simulink model "AXU5EV_Experiment_FOC"  (R2026b)
settings: Solver=FixedStepDiscrete  StopTime=.01  FixedStep=Ts_ACR
model workspace (MAT data in the model file):
  ADC_Calibration_Log2_N = 10
  ADC_Manual_Offset_Valid_A = 0
  ADC_Manual_Offset_Valid_B = 0
  Encoder_Counts_Per_Electrical_Period = 30000
  Encoder_Nanometres_Per_Count = 1000
  Experiment_Id_Limit_A = 0.5
  Experiment_Iq_Limit_A = 0.3
  Experiment_Parameter_Version = 20261117
  FOC_Fixed_Config.Version = 20261024
  FOC_Fixed_Config.Parameters.Rs = 1.45
  FOC_Fixed_Config.Parameters.Ld = 0.0118
  FOC_Fixed_Config.Parameters.Lq = 0.0118
  FOC_Fixed_Config.Parameters.psi = 0.0684240400279
  FOC_Fixed_Config.Parameters.Kp_ACR = 59
  FOC_Fixed_Config.Parameters.Ki_ACR = 7250
  FOC_Fixed_Config.Parameters.Kaw_d = 0.0122881355932
  FOC_Fixed_Config.Parameters.Kaw_q = 0.0122881355932
  FOC_Fixed_Config.Parameters.Ts_ACR = 0.0001
  FOC_Fixed_Config.Parameters.Udc = 48
  FOC_Fixed_Config.Fimath = embedded.fimath
  FOC_Fixed_Config.Fimath.RoundMode = 'convergent'
  FOC_Fixed_Config.Fimath.RoundingMethod = 'Convergent'
  FOC_Fixed_Config.Fimath.OverflowMode = 'saturate'
  FOC_Fixed_Config.Fimath.OverflowAction = 'Saturate'
  FOC_Fixed_Config.Fimath.ProductMode = 'FullPrecision'
  FOC_Fixed_Config.Fimath.SumMode = 'FullPrecision'
  FOC_Fixed_Config.Fimath.FixedOpFloatingYields = 'Fixed'
  FOC_Fixed_Config.Fimath.ProductWordLength = 32
  FOC_Fixed_Config.Fimath.SumWordLength = 32
  FOC_Fixed_Config.Fimath.MaxProductWordLength = 65535
  FOC_Fixed_Config.Fimath.MaxSumWordLength = 65535
  FOC_Fixed_Config.Fimath.ProductFractionLength = 30
  FOC_Fixed_Config.Fimath.ProductFixedExponent = -30
  FOC_Fixed_Config.Fimath.SumFractionLength = 30
  FOC_Fixed_Config.Fimath.SumFixedExponent = -30
  FOC_Fixed_Config.Fimath.SumSlopeAdjustmentFactor = 1
  FOC_Fixed_Config.Fimath.SumBias = 0
  FOC_Fixed_Config.Fimath.ProductSlopeAdjustmentFactor = 1
  FOC_Fixed_Config.Fimath.ProductBias = 0
  FOC_Fixed_Config.Fimath.CastBeforeSum = 1
  FOC_Fixed_Config.Fimath.SumSlope = 9.31322574615e-10
  FOC_Fixed_Config.Fimath.ProductSlope = 9.31322574615e-10
  FOC_Fixed_Config.Fimath.DDGMaxProductWordLength = 65535
  FOC_Fixed_Config.Fimath.DDGMaxSumWordLength = 65535
  FOC_Fixed_Config.Fimath.DDGProductFixedExponent = -30
  FOC_Fixed_Config.Fimath.DDGProductFractionLength = 30
  FOC_Fixed_Config.Fimath.DDGProductWordLength = 32
  FOC_Fixed_Config.Fimath.DDGSumFixedExponent = -30
  FOC_Fixed_Config.Fimath.DDGSumFractionLength = 30
  FOC_Fixed_Config.Fimath.DDGSumWordLength = 32
  FOC_Fixed_Config.Fimath.DDGProductBias = 0
  FOC_Fixed_Config.Fimath.DDGProductSlopeAdjustmentFactor = 1
  FOC_Fixed_Config.Fimath.DDGSumBias = 0
  FOC_Fixed_Config.Fimath.DDGSumSlopeAdjustmentFactor = 1
  FOC_Fixed_Config.Fimath.DDGCastBeforeSum = 1
  FOC_Fixed_Config.Fimath.DDGProductSlope = 9.31322574615e-10
  FOC_Fixed_Config.Fimath.DDGSumSlope = 9.31322574615e-10
  FOC_Fixed_Config.Types.Current = embedded.numerictype
  FOC_Fixed_Config.Types.Current.ReadOnly = 0
  FOC_Fixed_Config.Types.Current.Volatile = 0
  FOC_Fixed_Config.Types.Current.DataTypeMode = 'Fixed-point: binary point scaling'
  FOC_Fixed_Config.Types.Current.DataType = 'Fixed'
  FOC_Fixed_Config.Types.Current.Scaling = 'BinaryPoint'
  FOC_Fixed_Config.Types.Current.SignednessBool = 1
  FOC_Fixed_Config.Types.Current.Signedness = 'Signed'
  FOC_Fixed_Config.Types.Current.Signed = 1
  FOC_Fixed_Config.Types.Current.WordLength = 32
  FOC_Fixed_Config.Types.Current.FractionLength = 24
  FOC_Fixed_Config.Types.Current.BinaryPoint = 24
  FOC_Fixed_Config.Types.Current.Slope = 5.96046447754e-08
  FOC_Fixed_Config.Types.Current.FixedExponent = -24
  FOC_Fixed_Config.Types.Current.SlopeAdjustmentFactor = 1
  FOC_Fixed_Config.Types.Current.Bias = 0
  FOC_Fixed_Config.Types.Current.DataTypeOverride = 'Inherit'
  FOC_Fixed_Config.Types.Angle = embedded.numerictype
  FOC_Fixed_Config.Types.Angle.ReadOnly = 0
  FOC_Fixed_Config.Types.Angle.Volatile = 0
  FOC_Fixed_Config.Types.Angle.DataTypeMode = 'Fixed-point: binary point scaling'
  FOC_Fixed_Config.Types.Angle.DataType = 'Fixed'
  FOC_Fixed_Config.Types.Angle.Scaling = 'BinaryPoint'
  FOC_Fixed_Config.Types.Angle.SignednessBool = 1
  FOC_Fixed_Config.Types.Angle.Signedness = 'Signed'
  FOC_Fixed_Config.Types.Angle.Signed = 1
  FOC_Fixed_Config.Types.Angle.WordLength = 40
  FOC_Fixed_Config.Types.Angle.FractionLength = 32
  FOC_Fixed_Config.Types.Angle.BinaryPoint = 32
  FOC_Fixed_Config.Types.Angle.Slope = 2.32830643654e-10
  FOC_Fixed_Config.Types.Angle.FixedExponent = -32
  FOC_Fixed_Config.Types.Angle.SlopeAdjustmentFactor = 1
  FOC_Fixed_Config.Types.Angle.Bias = 0
  FOC_Fixed_Config.Types.Angle.DataTypeOverride = 'Inherit'
  FOC_Fixed_Config.Types.Omega = embedded.numerictype
  FOC_Fixed_Config.Types.Omega.ReadOnly = 0
  FOC_Fixed_Config.Types.Omega.Volatile = 0
  FOC_Fixed_Config.Types.Omega.DataTypeMode = 'Fixed-point: binary point scaling'
  FOC_Fixed_Config.Types.Omega.DataType = 'Fixed'
  FOC_Fixed_Config.Types.Omega.Scaling = 'BinaryPoint'
  FOC_Fixed_Config.Types.Omega.SignednessBool = 1
  FOC_Fixed_Config.Types.Omega.Signedness = 'Signed'
  FOC_Fixed_Config.Types.Omega.Signed = 1
  FOC_Fixed_Config.Types.Omega.WordLength = 40
  FOC_Fixed_Config.Types.Omega.FractionLength = 24
  FOC_Fixed_Config.Types.Omega.BinaryPoint = 24
  FOC_Fixed_Config.Types.Omega.Slope = 5.96046447754e-08
  FOC_Fixed_Config.Types.Omega.FixedExponent = -24
  FOC_Fixed_Config.Types.Omega.SlopeAdjustmentFactor = 1
  FOC_Fixed_Config.Types.Omega.Bias = 0
  FOC_Fixed_Config.Types.Omega.DataTypeOverride = 'Inherit'
  FOC_Fixed_Config.Types.Bus = embedded.numerictype
  FOC_Fixed_Config.Types.Bus.ReadOnly = 0
  FOC_Fixed_Config.Types.Bus.Volatile = 0
  FOC_Fixed_Config.Types.Bus.DataTypeMode = 'Fixed-point: binary point scaling'
  FOC_Fixed_Config.Types.Bus.DataType = 'Fixed'
  FOC_Fixed_Config.Types.Bus.Scaling = 'BinaryPoint'
  FOC_Fixed_Config.Types.Bus.SignednessBool = 0
  FOC_Fixed_Config.Types.Bus.Signedness = 'Unsigned'
  FOC_Fixed_Config.Types.Bus.Signed = 0
  FOC_Fixed_Config.Types.Bus.WordLength = 32
  FOC_Fixed_Config.Types.Bus.FractionLength = 24
  FOC_Fixed_Config.Types.Bus.BinaryPoint = 24
  FOC_Fixed_Config.Types.Bus.Slope = 5.96046447754e-08
  FOC_Fixed_Config.Types.Bus.FixedExponent = -24
  FOC_Fixed_Config.Types.Bus.SlopeAdjustmentFactor = 1
  FOC_Fixed_Config.Types.Bus.Bias = 0
  FOC_Fixed_Config.Types.Bus.DataTypeOverride = 'Inherit'
  FOC_Fixed_Config.Types.Work = embedded.numerictype
  FOC_Fixed_Config.Types.Work.ReadOnly = 0
  FOC_Fixed_Config.Types.Work.Volatile = 0
  FOC_Fixed_Config.Types.Work.DataTypeMode = 'Fixed-point: binary point scaling'
  FOC_Fixed_Config.Types.Work.DataType = 'Fixed'
  FOC_Fixed_Config.Types.Work.Scaling = 'BinaryPoint'
  FOC_Fixed_Config.Types.Work.SignednessBool = 1
  FOC_Fixed_Config.Types.Work.Signedness = 'Signed'
  FOC_Fixed_Config.Types.Work.Signed = 1
  FOC_Fixed_Config.Types.Work.WordLength = 64
  FOC_Fixed_Config.Types.Work.FractionLength = 40
  FOC_Fixed_Config.Types.Work.BinaryPoint = 40
  FOC_Fixed_Config.Types.Work.Slope = 9.09494701773e-13
  FOC_Fixed_Config.Types.Work.FixedExponent = -40
  FOC_Fixed_Config.Types.Work.SlopeAdjustmentFactor = 1
  FOC_Fixed_Config.Types.Work.Bias = 0
  FOC_Fixed_Config.Types.Work.DataTypeOverride = 'Inherit'
  FOC_Fixed_Config.Types.Square = embedded.numerictype
  FOC_Fixed_Config.Types.Square.ReadOnly = 0
  FOC_Fixed_Config.Types.Square.Volatile = 0
  FOC_Fixed_Config.Types.Square.DataTypeMode = 'Fixed-point: binary point scaling'
  FOC_Fixed_Config.Types.Square.DataType = 'Fixed'
  FOC_Fixed_Config.Types.Square.Scaling = 'BinaryPoint'
  FOC_Fixed_Config.Types.Square.SignednessBool = 0
  FOC_Fixed_Config.Types.Square.Signedness = 'Unsigned'
  FOC_Fixed_Config.Types.Square.Signed = 0
  FOC_Fixed_Config.Types.Square.WordLength = 64
  FOC_Fixed_Config.Types.Square.FractionLength = 36
  FOC_Fixed_Config.Types.Square.BinaryPoint = 36
  FOC_Fixed_Config.Types.Square.Slope = 1.45519152284e-11
  FOC_Fixed_Config.Types.Square.FixedExponent = -36
  FOC_Fixed_Config.Types.Square.SlopeAdjustmentFactor = 1
  FOC_Fixed_Config.Types.Square.Bias = 0
  FOC_Fixed_Config.Types.Square.DataTypeOverride = 'Inherit'
  FOC_Fixed_Config.Types.DivideWide = embedded.numerictype
  FOC_Fixed_Config.Types.DivideWide.ReadOnly = 0
  FOC_Fixed_Config.Types.DivideWide.Volatile = 0
  FOC_Fixed_Config.Types.DivideWide.DataTypeMode = 'Fixed-point: binary point scaling'
  FOC_Fixed_Config.Types.DivideWide.DataType = 'Fixed'
  FOC_Fixed_Config.Types.DivideWide.Scaling = 'BinaryPoint'
  FOC_Fixed_Config.Types.DivideWide.SignednessBool = 0
  FOC_Fixed_Config.Types.DivideWide.Signedness = 'Unsigned'
  FOC_Fixed_Config.Types.DivideWide.Signed = 0
  FOC_Fixed_Config.Types.DivideWide.WordLength = 72
  FOC_Fixed_Config.Types.DivideWide.FractionLength = 40
  FOC_Fixed_Config.Types.DivideWide.BinaryPoint = 40
  FOC_Fixed_Config.Types.DivideWide.Slope = 9.09494701773e-13
  FOC_Fixed_Config.Types.DivideWide.FixedExponent = -40
  FOC_Fixed_Config.Types.DivideWide.SlopeAdjustmentFactor = 1
  FOC_Fixed_Config.Types.DivideWide.Bias = 0
  FOC_Fixed_Config.Types.DivideWide.DataTypeOverride = 'Inherit'
  FOC_Fixed_Config.Types.Duty = embedded.numerictype
  FOC_Fixed_Config.Types.Duty.ReadOnly = 0
  FOC_Fixed_Config.Types.Duty.Volatile = 0
  FOC_Fixed_Config.Types.Duty.DataTypeMode = 'Fixed-point: binary point scaling'
  FOC_Fixed_Config.Types.Duty.DataType = 'Fixed'
  FOC_Fixed_Config.Types.Duty.Scaling = 'BinaryPoint'
  FOC_Fixed_Config.Types.Duty.SignednessBool = 0
  FOC_Fixed_Config.Types.Duty.Signedness = 'Unsigned'
  FOC_Fixed_Config.Types.Duty.Signed = 0
  FOC_Fixed_Config.Types.Duty.WordLength = 32
  FOC_Fixed_Config.Types.Duty.FractionLength = 30
  FOC_Fixed_Config.Types.Duty.BinaryPoint = 30
  FOC_Fixed_Config.Types.Duty.Slope = 9.31322574615e-10
  FOC_Fixed_Config.Types.Duty.FixedExponent = -30
  FOC_Fixed_Config.Types.Duty.SlopeAdjustmentFactor = 1
  FOC_Fixed_Config.Types.Duty.Bias = 0
  FOC_Fixed_Config.Types.Duty.DataTypeOverride = 'Inherit'
  FOC_Fixed_Config.Types.Coefficient = embedded.numerictype
  FOC_Fixed_Config.Types.Coefficient.ReadOnly = 0
  FOC_Fixed_Config.Types.Coefficient.Volatile = 0
  FOC_Fixed_Config.Types.Coefficient.DataTypeMode = 'Fixed-point: binary point scaling'
  FOC_Fixed_Config.Types.Coefficient.DataType = 'Fixed'
  FOC_Fixed_Config.Types.Coefficient.Scaling = 'BinaryPoint'
  FOC_Fixed_Config.Types.Coefficient.SignednessBool = 1
  FOC_Fixed_Config.Types.Coefficient.Signedness = 'Signed'
  FOC_Fixed_Config.Types.Coefficient.Signed = 1
  FOC_Fixed_Config.Types.Coefficient.WordLength = 64
  FOC_Fixed_Config.Types.Coefficient.FractionLength = 40
  FOC_Fixed_Config.Types.Coefficient.BinaryPoint = 40
  FOC_Fixed_Config.Types.Coefficient.Slope = 9.09494701773e-13
  FOC_Fixed_Config.Types.Coefficient.FixedExponent = -40
  FOC_Fixed_Config.Types.Coefficient.SlopeAdjustmentFactor = 1
  FOC_Fixed_Config.Types.Coefficient.Bias = 0
  FOC_Fixed_Config.Types.Coefficient.DataTypeOverride = 'Inherit'
  FOC_Fixed_Config.Types.Time = embedded.numerictype
  FOC_Fixed_Config.Types.Time.ReadOnly = 0
  FOC_Fixed_Config.Types.Time.Volatile = 0
  FOC_Fixed_Config.Types.Time.DataTypeMode = 'Fixed-point: binary point scaling'
  FOC_Fixed_Config.Types.Time.DataType = 'Fixed'
  FOC_Fixed_Config.Types.Time.Scaling = 'BinaryPoint'
  FOC_Fixed_Config.Types.Time.SignednessBool = 1
  FOC_Fixed_Config.Types.Time.Signedness = 'Signed'
  FOC_Fixed_Config.Types.Time.Signed = 1
  FOC_Fixed_Config.Types.Time.WordLength = 64
  FOC_Fixed_Config.Types.Time.FractionLength = 40
  FOC_Fixed_Config.Types.Time.BinaryPoint = 40
  FOC_Fixed_Config.Types.Time.Slope = 9.09494701773e-13
  FOC_Fixed_Config.Types.Time.FixedExponent = -40
  FOC_Fixed_Config.Types.Time.SlopeAdjustmentFactor = 1
  FOC_Fixed_Config.Types.Time.Bias = 0
  FOC_Fixed_Config.Types.Time.DataTypeOverride = 'Inherit'
  FOC_Fixed_Config.Types.Reset = 'boolean'
  FOC_Fixed_Config.Types.Sector = 'uint8'
  FOC_Fixed_Config.TypeStrings.Current = 'fixdt(1,32,24)'
  FOC_Fixed_Config.TypeStrings.Angle = 'fixdt(1,40,32)'
  FOC_Fixed_Config.TypeStrings.Omega = 'fixdt(1,40,24)'
  FOC_Fixed_Config.TypeStrings.Bus = 'fixdt(0,32,24)'
  FOC_Fixed_Config.TypeStrings.Work = 'fixdt(1,64,40)'
  FOC_Fixed_Config.TypeStrings.Square = 'fixdt(0,64,36)'
  FOC_Fixed_Config.TypeStrings.DivideWide = 'fixdt(0,72,40)'
  FOC_Fixed_Config.TypeStrings.Duty = 'fixdt(0,32,30)'
  FOC_Fixed_Config.TypeStrings.Coefficient = 'fixdt(1,64,40)'
  FOC_Fixed_Config.TypeStrings.Time = 'fixdt(1,64,40)'
  FOC_Fixed_Config.TypeStrings.Reset = 'boolean'
  FOC_Fixed_Config.TypeStrings.Sector = 'uint8'
  FOC_Fixed_Config.Ranges.phase_current_A = 2
  FOC_Fixed_Config.Ranges.reference_A = 2
  FOC_Fixed_Config.Ranges.theta_abs_rad = 25.1327412287
  FOC_Fixed_Config.Ranges.omega_abs_radps = 100
  FOC_Fixed_Config.Ranges.Vdc_min_V = 12
  FOC_Fixed_Config.Ranges.Vdc_max_V = 60
  FOC_Fixed_Config.Ranges.verified_duration_s = 60
  FOC_Fixed_Config.Ranges.state_initial_V = 0
  FOC_Fixed_Config.Ranges.scope = 'engineering verification envelope, not motor/drive ratings'
  FOC_Fixed_Config.Ranges.park_axis_bound_A = 3.52766841475
  FOC_Fixed_Config.Ranges.error_bound_A = 5.52766841475
  FOC_Fixed_Config.Ranges.feedforward_bound_V = 11.0050527322
  FOC_Fixed_Config.Ranges.integrator_bound_V = 703.086461988
  FOC_Fixed_Config.Ranges.raw_voltage_bound_V = 1040.22395119
  FOC_Fixed_Config.Ranges.square_sum_bound_V2 = 2164131.73726
  FOC_Fixed_Config.Coefficients.Kp.original = 59
  FOC_Fixed_Config.Coefficients.Kp.quantized = 59
  FOC_Fixed_Config.Coefficients.Kp.error = -1.42108547152e-14
  FOC_Fixed_Config.Coefficients.KiTs.original = 0.725
  FOC_Fixed_Config.Coefficients.KiTs.quantized = 0.725
  FOC_Fixed_Config.Coefficients.KiTs.error = 3.63709062867e-13
  FOC_Fixed_Config.Coefficients.Kaw_d.original = 0.0122881355932
  FOC_Fixed_Config.Coefficients.Kaw_d.quantized = 0.0122881355928
  FOC_Fixed_Config.Coefficients.Kaw_d.error = -3.94628774103e-13
  FOC_Fixed_Config.Coefficients.Kaw_q.original = 0.0122881355932
  FOC_Fixed_Config.Coefficients.Kaw_q.quantized = 0.0122881355928
  FOC_Fixed_Config.Coefficients.Kaw_q.error = -3.94628774103e-13
  FOC_Fixed_Config.Coefficients.Ld.original = 0.0118
  FOC_Fixed_Config.Coefficients.Ld.quantized = 0.0118000000002
  FOC_Fixed_Config.Coefficients.Ld.error = 2.21189386251e-13
  FOC_Fixed_Config.Coefficients.Lq.original = 0.0118
  FOC_Fixed_Config.Coefficients.Lq.quantized = 0.0118000000002
  FOC_Fixed_Config.Coefficients.Lq.error = 2.21189386251e-13
  FOC_Fixed_Config.Coefficients.psi.original = 0.0684240400279
  FOC_Fixed_Config.Coefficients.psi.quantized = 0.0684240400278
  FOC_Fixed_Config.Coefficients.psi.error = -1.18724474696e-13
  FOC_Fixed_Config.Coefficients.Ts.original = 0.0001
  FOC_Fixed_Config.Coefficients.Ts.quantized = 0.000100000000202
  FOC_Fixed_Config.Coefficients.Ts.error = 2.02271616882e-13
  FOC_Fixed_Config.Coefficients.InvSqrt3.original = 0.57735026919
  FOC_Fixed_Config.Coefficients.InvSqrt3.quantized = 0.57735026919
  FOC_Fixed_Config.Coefficients.InvSqrt3.error = 3.66262575824e-13
  FOC_Fixed_Config.Coefficients.TwoThird.original = 0.666666666667
  FOC_Fixed_Config.Coefficients.TwoThird.quantized = 0.666666666667
  FOC_Fixed_Config.Coefficients.TwoThird.error = 3.03201908025e-13
  FOC_Fixed_Config.Coefficients.C0866.original = 0.866
  FOC_Fixed_Config.Coefficients.C0866.quantized = 0.866
  FOC_Fixed_Config.Coefficients.C0866.error = -1.45439216226e-14
  FOC_Fixed_Config.Coefficients.C17321.original = 1.7321
  FOC_Fixed_Config.Coefficients.C17321.quantized = 1.7321
  FOC_Fixed_Config.Coefficients.C17321.error = 1.73194791842e-13
  FOC_Fixed_Config.Coefficients.C09.original = 0.9
  FOC_Fixed_Config.Coefficients.C09.quantized = 0.9
  FOC_Fixed_Config.Coefficients.C09.error = -3.6382008517e-13
  FOC_Fixed_Config.Coefficients.C0999.original = 0.999
  FOC_Fixed_Config.Coefficients.C0999.quantized = 0.999
  FOC_Fixed_Config.Coefficients.C0999.error = -2.03725925019e-13
  FOC_Fixed_Config.Coefficients.Epsilon.original = 1e-06
  FOC_Fixed_Config.Coefficients.Epsilon.quantized = 1.00000033854e-06
  FOC_Fixed_Config.Coefficients.Epsilon.error = 3.38535755918e-13
  FOC_Fixed_Config.Coefficients.DutyGain.original = -20000
  FOC_Fixed_Config.Coefficients.DutyGain.quantized = -20000
  FOC_Fixed_Config.Coefficients.DutyGain.error = 0
  FOC_Fixed_Parameters.Rs = 1.45
  FOC_Fixed_Parameters.Ld = 0.0118
  FOC_Fixed_Parameters.Lq = 0.0118
  FOC_Fixed_Parameters.psi = 0.0684240400279
  FOC_Fixed_Parameters.Kp_ACR = 59
  FOC_Fixed_Parameters.Ki_ACR = 7250
  FOC_Fixed_Parameters.Kaw_d = 0.0122881355932
  FOC_Fixed_Parameters.Kaw_q = 0.0122881355932
  FOC_Fixed_Parameters.Ts_ACR = 0.0001
  FOC_Fixed_Parameters.Udc = 48
  Feedback_Id_Step = 500
  Feedback_Tick_Hz = 50000000
  Feedback_Tick_Step = 5000
  Grating_Resolution_mm_per_count = 0.001
  Hardware_Binding_Complete = 0
  Hold_Ticks = 30000
  Host_AutoStart_EN = 0
  Host_Load_N = 0
  Host_Ready_Ticks = 5
  Host_Speed_Ramp_s = 0.2
  Host_Start_s = 0.05
  Host_Traj_Amax = 200
  Host_Traj_Jmax = 1000
  Host_Traj_Vmax = 20
  Id_Init_Step = 5e-05
  Id_Init_Target = 0.5
  Id_Release_Ramp_Ticks = 2000
  Iq_fric_run = 0.05
  Iq_fric_start = 0.4
  Iq_int_limit = 0.2
  Kaw_d = 0.0122881355932
  Kaw_q = 0.0122881355932
  Kaw_s = 0.4
  Ki_ACR = 7250
  Ki_ASR = 0.05
  Kp_ACR = 59
  Kp_ASR = 0.03
  Kp_pos = 5
  PMLSM_Kf_peak_N_per_Apeak = 21.4960461481
  PMLSM_Ld_H = 0.0118
  PMLSM_Lq_H = 0.0118
  PMLSM_Rs_ohm = 1.45
  PMLSM_psi_f_Wb = 0.0684240400279
  PMLSM_tau_NN_m = 0.03
  Physical_Calibration_Valid = 0
  Pos_deadband = 0.02
  Ramp_Ticks = 10000
  Speed_loop_Iq_Limit = 0.3
  Tau_e_mm = 30
  Theta_Offset_Fine = 0
  Total_Moving_Mass_Known = 0
  Total_Moving_Mass_kg = nan
  Ts = 0.0001
  Ts_ACR = 0.0001
  Ts_ASR = 0.001
  Ts_POS = 0.01
  Tuning_Current_Xi = 0.707106781187
  Udc = 48
  V_meas_max = 500
  V_pos_max_mmps = 20
  X_max_hard = 120
  X_max_soft = 110
  X_min_hard = -120
  X_min_soft = -110
  delay_N = 50
  theta_align_const = 0
  v_ff_eps = 0.5
  v_meas_zero_eps = 0.5
  v_over_eps = 3
  v_ref_max = 20
  v_ref_set_rate_dn = 100
  v_ref_set_rate_up = 100
  v_ref_set_step_dn = 0.01
  v_ref_set_step_up = 0.01
  v_ref_zero_eps = 0
libraries: mcbeeMathTransformLib x2, simulink x2
settings Model: DataTypeOverride=Off  Creator=lww  LastModifiedBy=lww
settings OptimizationCC: DefaultParameterBehavior=Inlined
settings DebuggingCC: FixptConstOverflowMsg=error  IntegerOverflowMsg=error  IntegerSaturationMsg=error

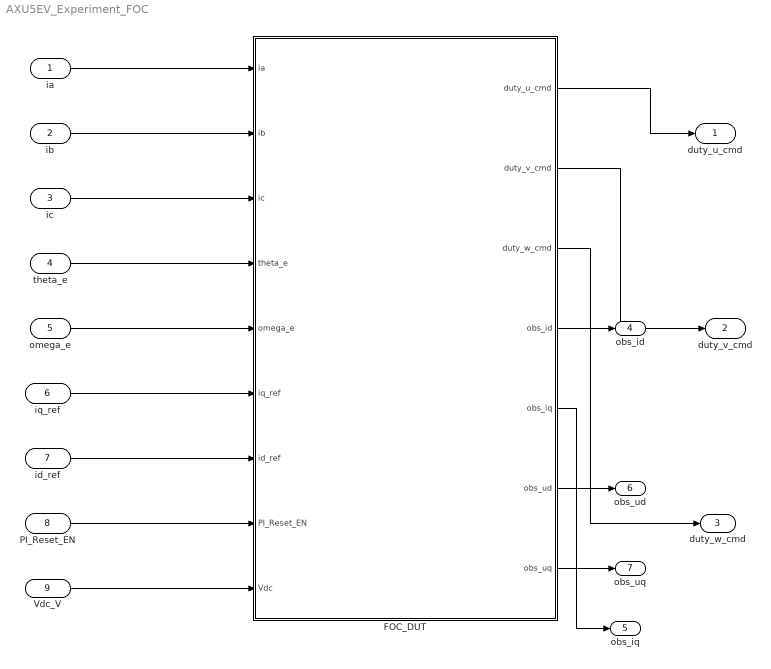
== system AXU5EV_Experiment_FOC ==
  ia : Inport  OutDataTypeStr=FOC_Fixed_Config.Types.Current  SampleTime=Ts_ACR  Interpolate=off
  ib : Inport  Port=2  OutDataTypeStr=FOC_Fixed_Config.Types.Current  SampleTime=Ts_ACR  Interpolate=off
  ic : Inport  Port=3  OutDataTypeStr=FOC_Fixed_Config.Types.Current  SampleTime=Ts_ACR  Interpolate=off
  theta_e : Inport  Port=4  OutDataTypeStr=FOC_Fixed_Config.Types.Angle  SampleTime=Ts_ACR  Interpolate=off
  omega_e : Inport  Port=5  OutDataTypeStr=FOC_Fixed_Config.Types.Omega  SampleTime=Ts_ACR  Interpolate=off
  iq_ref : Inport  Port=6  OutDataTypeStr=FOC_Fixed_Config.Types.Current  SampleTime=Ts_ACR  Interpolate=off
  id_ref : Inport  Port=7  OutDataTypeStr=FOC_Fixed_Config.Types.Current  SampleTime=Ts_ACR  Interpolate=off
  PI_Reset_EN : Inport  Port=8  OutDataTypeStr=boolean  SampleTime=Ts_ACR  Interpolate=off
  Vdc_V : Inport  Port=9  OutDataTypeStr=FOC_Fixed_Config.Types.Bus  SampleTime=Ts_ACR  Interpolate=off
  FOC_DUT : Subsystem  TreatAsAtomicUnit=on
  duty_u_cmd : Outport  OutDataTypeStr=FOC_Fixed_Config.Types.Duty
  duty_v_cmd : Outport  Port=2  OutDataTypeStr=FOC_Fixed_Config.Types.Duty
  duty_w_cmd : Outport  Port=3  OutDataTypeStr=FOC_Fixed_Config.Types.Duty
  obs_id : Outport  Port=4
  obs_iq : Outport  Port=5
  obs_ud : Outport  Port=6
  obs_uq : Outport  Port=7
  wires:
  ia/1 -> FOC_DUT/1(ia)
  ib/1 -> FOC_DUT/2(ib)
  ic/1 -> FOC_DUT/3(ic)
  theta_e/1 -> FOC_DUT/4(theta_e)
  omega_e/1 -> FOC_DUT/5(omega_e)
  iq_ref/1 -> FOC_DUT/6(iq_ref)
  id_ref/1 -> FOC_DUT/7(id_ref)
  PI_Reset_EN/1 -> FOC_DUT/8(PI_Reset_EN)
  FOC_DUT/1(duty_u_cmd) -> duty_u_cmd/1
  FOC_DUT/2(duty_v_cmd) -> duty_v_cmd/1
  FOC_DUT/3(duty_w_cmd) -> duty_w_cmd/1
  Vdc_V/1 -> FOC_DUT/9(Vdc)
  FOC_DUT/7(obs_uq) -> obs_uq/1
  FOC_DUT/6(obs_ud) -> obs_ud/1
  FOC_DUT/5(obs_iq) -> obs_iq/1
  FOC_DUT/4(obs_id) -> obs_id/1

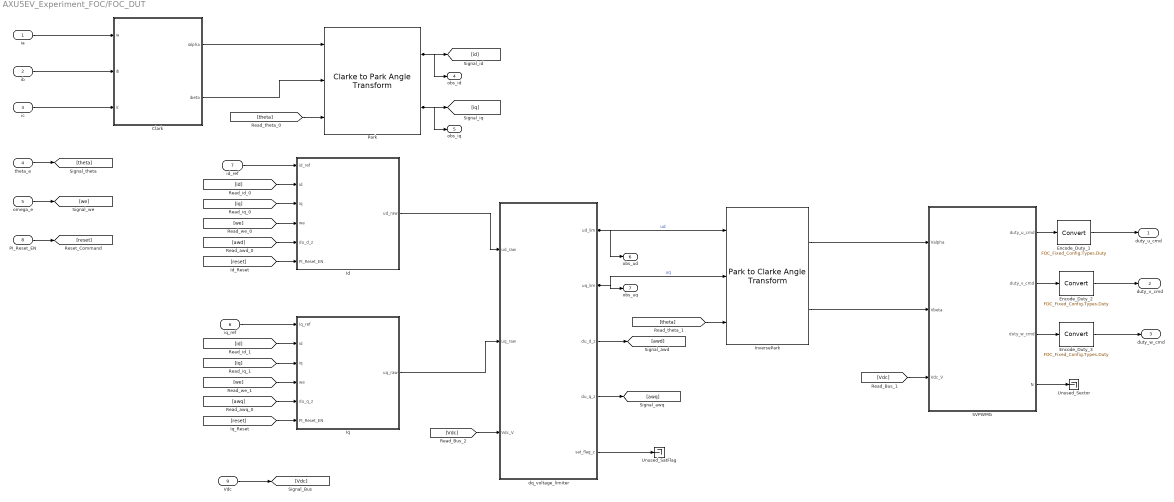
== system AXU5EV_Experiment_FOC/FOC_DUT ==
  ia : Inport
  ib : Inport  Port=2
  ic : Inport  Port=3
  theta_e : Inport  Port=4
  omega_e : Inport  Port=5
  iq_ref : Inport  Port=6
  id_ref : Inport  Port=7
  PI_Reset_EN : Inport  Port=8
  Vdc : Inport  Port=9
  Clark : Subsystem  TreatAsAtomicUnit=on  RTWFcnName=Clack_Fun
      settings: RTWFcnNameOpts=User specified
  Encode_Duty_1 : DataTypeConversion  OutDataTypeStr=FOC_Fixed_Config.Types.Duty  RndMeth=Convergent
  Encode_Duty_2 : DataTypeConversion  OutDataTypeStr=FOC_Fixed_Config.Types.Duty  RndMeth=Convergent
  Encode_Duty_3 : DataTypeConversion  OutDataTypeStr=FOC_Fixed_Config.Types.Duty  RndMeth=Convergent
  Id : Subsystem  TreatAsAtomicUnit=on  RTWFcnName=Id_Fun
      settings: RTWFcnNameOpts=User specified
  InversePark : mcbeeMathTransformLib/Park to Clarke Angle Transform  AxisAlignment=D-axis  UseWithEmbedded=on  PhaseInput=Two inputs  ThetaInput=Electrical position  AngleInput=Radians  N_points=1024
      settings: LibrarySourceBlock=mcbhdllib/Controls/Math Transforms/Inverse Park Transform
  Iq : Subsystem  TreatAsAtomicUnit=on  RTWFcnName=Iq_Fun
      settings: RTWFcnNameOpts=User specified
  Park : mcbeeMathTransformLib/Clarke to Park Angle Transform  AxisAlignment=D-axis  UseWithEmbedded=on  PhaseInput=Two inputs  ThetaInput=Electrical position  AngleInput=Radians  N_points=1024
      settings: LibrarySourceBlock=mcblib/Controls/Math Transforms/Park Transform
  SVPWMG : Subsystem  TreatAsAtomicUnit=on  RTWFcnName=SVPWM_Gen_Fun
      settings: RTWFcnNameOpts=User specified
  Unused_SatFlag : Terminator
  Unused_Sector : Terminator
  dq_voltage_limiter : Subsystem
  duty_u_cmd : Outport
  duty_v_cmd : Outport  Port=2
  duty_w_cmd : Outport  Port=3
  obs_id : Outport  Port=4
  obs_iq : Outport  Port=5
  obs_ud : Outport  Port=6
  obs_uq : Outport  Port=7
  wires:
  ia/1 -> Clark/1(ia)
  ib/1 -> Clark/2(ib)
  ic/1 -> Clark/3(ic)
  theta_e/1 -> [theta]
  omega_e/1 -> [we]
  iq_ref/1 -> Iq/1(Iq_ref)
  id_ref/1 -> Id/1(id_ref)
  PI_Reset_EN/1 -> [reset]
  Vdc/1 -> [Vdc]
  Clark/1(ialpha) -> Park/1
  Clark/2(ibeta) -> Park/2
  Encode_Duty_1/1 -> duty_u_cmd/1
  Encode_Duty_2/1 -> duty_v_cmd/1
  Encode_Duty_3/1 -> duty_w_cmd/1
  Id/1(ud_raw) -> dq_voltage_limiter/1(ud_raw)
  [reset] -> Id/6(PI_Reset_EN)
  InversePark/1 -> SVPWMG/1(Valpha)
  InversePark/2 -> SVPWMG/2(Vbeta)
  Iq/1(uq_raw) -> dq_voltage_limiter/2(uq_raw)
  [reset] -> Iq/6(PI_Reset_EN)
  [Vdc] -> SVPWMG/3(Vdc_V)
  [Vdc] -> dq_voltage_limiter/3(Vdc_V)
  [awd] -> Id/5(du_d_z)
  [awq] -> Iq/5(du_q_z)
  [id] -> Id/2(id)
  [id] -> Iq/2(id)
  [iq] -> Id/3(iq)
  [iq] -> Iq/3(iq)
  [theta] -> Park/3
  [theta] -> InversePark/3
  [we] -> Id/4(we)
  [we] -> Iq/4(we)
  SVPWMG/1(duty_u_cmd) -> Encode_Duty_1/1
  SVPWMG/2(duty_v_cmd) -> Encode_Duty_2/1
  SVPWMG/3(duty_w_cmd) -> Encode_Duty_3/1
  SVPWMG/4("N ") -> Unused_Sector/1
  dq_voltage_limiter/4(du_q_z) -> [awq]
  dq_voltage_limiter/5(sat_flag_z) -> Unused_SatFlag/1
  dq_voltage_limiter/3(du_d_z) -> [awd]
  dq_voltage_limiter/2(uq_lim) -> InversePark/2, obs_uq/1  "uq"
  dq_voltage_limiter/1(ud_lim) -> obs_ud/1, InversePark/1  "ud"
  Park/2 -> obs_iq/1, [iq]
  Park/1 -> obs_id/1, [id]

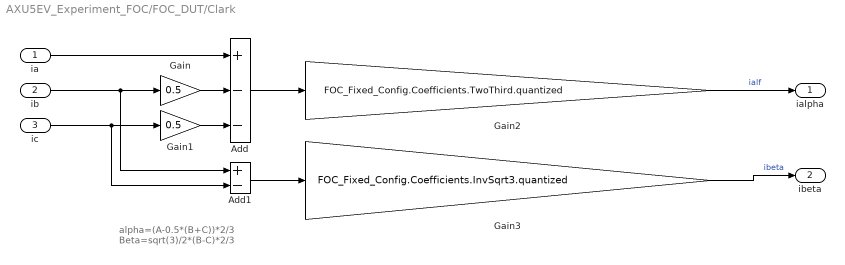
== system AXU5EV_Experiment_FOC/FOC_DUT/Clark ==
  note: alpha=(A-0.5*(B+C))*2/3
      | Beta=sqrt(3)/2*(B-C)*2/3
  ia : Inport
  ib : Inport  Port=2
  ic : Inport  Port=3
  Add : Sum  Inputs=+--  OutDataTypeStr=FOC_Fixed_Config.Types.Work  AccumDataTypeStr=FOC_Fixed_Config.Types.Work  RndMeth=Convergent  SaturateOnIntegerOverflow=on
  Add1 : Sum  Inputs=+-  OutDataTypeStr=FOC_Fixed_Config.Types.Work  AccumDataTypeStr=FOC_Fixed_Config.Types.Work  RndMeth=Convergent  SaturateOnIntegerOverflow=on
  Gain : Gain  Gain=0.5  ParamDataTypeStr=FOC_Fixed_Config.Types.Coefficient  OutDataTypeStr=FOC_Fixed_Config.Types.Work  RndMeth=Convergent  SaturateOnIntegerOverflow=on
  Gain1 : Gain  Gain=0.5  ParamDataTypeStr=FOC_Fixed_Config.Types.Coefficient  OutDataTypeStr=FOC_Fixed_Config.Types.Work  RndMeth=Convergent  SaturateOnIntegerOverflow=on
  Gain2 : Gain  Gain=FOC_Fixed_Config.Coefficients.TwoThird.quantized  ParamDataTypeStr=FOC_Fixed_Config.Types.Coefficient  OutDataTypeStr=FOC_Fixed_Config.Types.Work  RndMeth=Convergent  SaturateOnIntegerOverflow=on
  Gain3 : Gain  Gain=FOC_Fixed_Config.Coefficients.InvSqrt3.quantized  ParamDataTypeStr=FOC_Fixed_Config.Types.Coefficient  OutDataTypeStr=FOC_Fixed_Config.Types.Work  RndMeth=Convergent  SaturateOnIntegerOverflow=on
  ialpha : Outport
  ibeta : Outport  Port=2
  wires:
  Gain1/1 -> Add/3
  ia/1 -> Add/1
  ib/1 -> Add1/1, Gain/1
  Add1/1 -> Gain3/1
  ic/1 -> Add1/2, Gain1/1
  Gain3/1 -> ibeta/1  "ibeta"
  Add/1 -> Gain2/1
  Gain2/1 -> ialpha/1  "ialf"
  Gain/1 -> Add/2

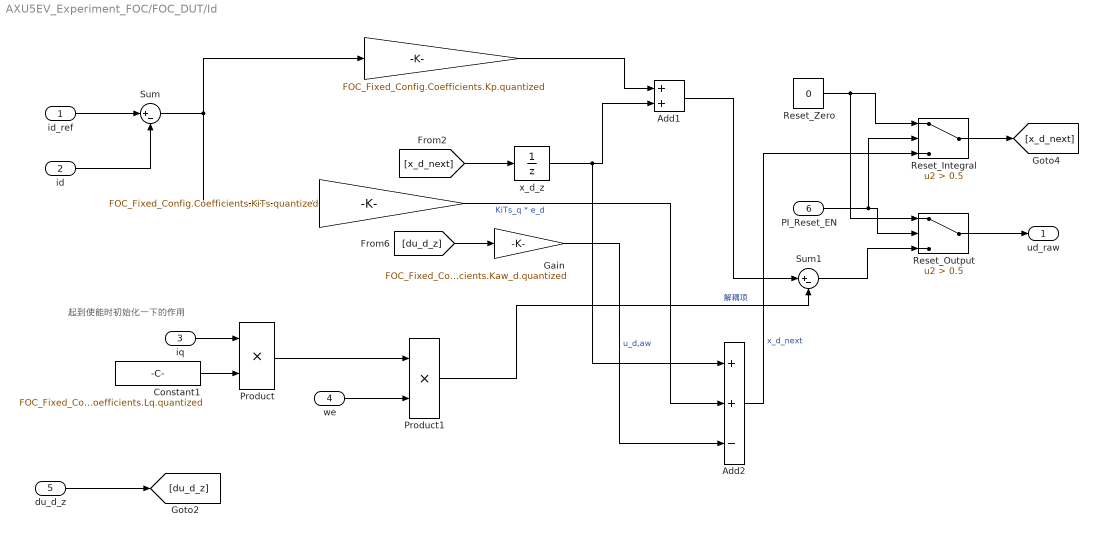
== system AXU5EV_Experiment_FOC/FOC_DUT/Id ==
  note: 起到使能时初始化一下的作用
  id_ref : Inport
  id : Inport  Port=2
  iq : Inport  Port=3
  we : Inport  Port=4
  du_d_z : Inport  Port=5
  PI_Reset_EN : Inport  Port=6
  " " : Gain  Gain=FOC_Fixed_Config.Coefficients.KiTs.quantized  ParamDataTypeStr=FOC_Fixed_Config.Types.Coefficient  OutDataTypeStr=FOC_Fixed_Config.Types.Work  RndMeth=Convergent  SaturateOnIntegerOverflow=on
  "  " : Gain  Gain=FOC_Fixed_Config.Coefficients.Kp.quantized  ParamDataTypeStr=FOC_Fixed_Config.Types.Coefficient  OutDataTypeStr=FOC_Fixed_Config.Types.Work  RndMeth=Convergent  SaturateOnIntegerOverflow=on
  Add1 : Sum  OutDataTypeStr=FOC_Fixed_Config.Types.Work  AccumDataTypeStr=FOC_Fixed_Config.Types.Work  RndMeth=Convergent  SaturateOnIntegerOverflow=on
  Add2 : Sum  Inputs=++-  OutDataTypeStr=FOC_Fixed_Config.Types.Work  AccumDataTypeStr=FOC_Fixed_Config.Types.Work  RndMeth=Convergent  SaturateOnIntegerOverflow=on
  Constant1 : Constant  Value=FOC_Fixed_Config.Coefficients.Lq.quantized  OutDataTypeStr=FOC_Fixed_Config.Types.Work
  Gain : Gain  Gain=FOC_Fixed_Config.Coefficients.Kaw_d.quantized  ParamDataTypeStr=FOC_Fixed_Config.Types.Coefficient  OutDataTypeStr=FOC_Fixed_Config.Types.Work  RndMeth=Convergent  SaturateOnIntegerOverflow=on
  Product : Product  OutDataTypeStr=FOC_Fixed_Config.Types.Work  RndMeth=Convergent  SaturateOnIntegerOverflow=on
  Product1 : Product  OutDataTypeStr=FOC_Fixed_Config.Types.Work  RndMeth=Convergent  SaturateOnIntegerOverflow=on
  Reset_Integral : Switch  Criteria=u2 > Threshold  Threshold=0.5  OutDataTypeStr=FOC_Fixed_Config.Types.Work  RndMeth=Convergent  InputSameDT=off
  Reset_Output : Switch  Criteria=u2 > Threshold  Threshold=0.5  OutDataTypeStr=FOC_Fixed_Config.Types.Work  RndMeth=Convergent  InputSameDT=off
  Reset_Zero : Constant  Value=0  OutDataTypeStr=FOC_Fixed_Config.Types.Work
  Sum : Sum  Inputs=|+-  OutDataTypeStr=FOC_Fixed_Config.Types.Work  AccumDataTypeStr=FOC_Fixed_Config.Types.Work  RndMeth=Convergent  SaturateOnIntegerOverflow=on
  Sum1 : Sum  Inputs=|+-  OutDataTypeStr=FOC_Fixed_Config.Types.Work  AccumDataTypeStr=FOC_Fixed_Config.Types.Work  RndMeth=Convergent  SaturateOnIntegerOverflow=on
  x_d_z : UnitDelay  SampleTime=-1
  ud_raw : Outport
  wires:
  Product1/1 -> Sum1/2  "解耦项"
  Add1/1 -> Sum1/1
  x_d_z/1 -> Add1/2, Add2/1
  Gain/1 -> Add2/3  "u_d,aw"
  " "/1 -> Add2/2  "KiTs_q * e_d"
  Sum1/1 -> Reset_Output/3
  Add2/1 -> Reset_Integral/3  "x_d_next"
  Reset_Zero/1 -> Reset_Integral/1, Reset_Output/1
  PI_Reset_EN/1 -> Reset_Integral/2, Reset_Output/2
  Reset_Integral/1 -> [x_d_next]
  Reset_Output/1 -> ud_raw/1
  iq/1 -> Product/1
  id_ref/1 -> Sum/1
  id/1 -> Sum/2
  Sum/1 -> " "/1, "  "/1
  we/1 -> Product1/2
  Product/1 -> Product1/1
  Constant1/1 -> Product/2
  "  "/1 -> Add1/1
  du_d_z/1 -> [du_d_z]
  [x_d_next] -> x_d_z/1
  [du_d_z] -> Gain/1

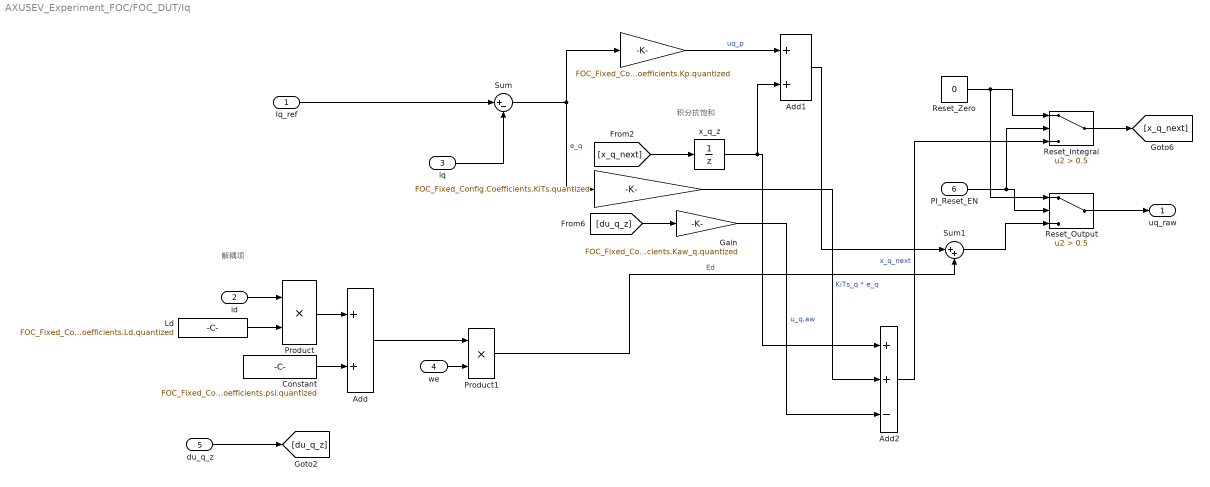
== system AXU5EV_Experiment_FOC/FOC_DUT/Iq ==
  note: 解耦项
  note: 积分抗饱和
  Iq_ref : Inport
  id : Inport  Port=2
  iq : Inport  Port=3
  we : Inport  Port=4
  du_q_z : Inport  Port=5
  PI_Reset_EN : Inport  Port=6
  " " : Gain  Gain=FOC_Fixed_Config.Coefficients.KiTs.quantized  ParamDataTypeStr=FOC_Fixed_Config.Types.Coefficient  OutDataTypeStr=FOC_Fixed_Config.Types.Work  RndMeth=Convergent  SaturateOnIntegerOverflow=on
  "  " : Gain  Gain=FOC_Fixed_Config.Coefficients.Kp.quantized  ParamDataTypeStr=FOC_Fixed_Config.Types.Coefficient  OutDataTypeStr=FOC_Fixed_Config.Types.Work  RndMeth=Convergent  SaturateOnIntegerOverflow=on
  Add : Sum  OutDataTypeStr=FOC_Fixed_Config.Types.Work  AccumDataTypeStr=FOC_Fixed_Config.Types.Work  RndMeth=Convergent  SaturateOnIntegerOverflow=on
  Add1 : Sum  OutDataTypeStr=FOC_Fixed_Config.Types.Work  AccumDataTypeStr=FOC_Fixed_Config.Types.Work  RndMeth=Convergent  SaturateOnIntegerOverflow=on
  Add2 : Sum  Inputs=++-  OutDataTypeStr=FOC_Fixed_Config.Types.Work  AccumDataTypeStr=FOC_Fixed_Config.Types.Work  RndMeth=Convergent  SaturateOnIntegerOverflow=on
  Constant : Constant  Value=FOC_Fixed_Config.Coefficients.psi.quantized  OutDataTypeStr=FOC_Fixed_Config.Types.Work
  Gain : Gain  Gain=FOC_Fixed_Config.Coefficients.Kaw_q.quantized  ParamDataTypeStr=FOC_Fixed_Config.Types.Coefficient  OutDataTypeStr=FOC_Fixed_Config.Types.Work  RndMeth=Convergent  SaturateOnIntegerOverflow=on
  Ld : Constant  Value=FOC_Fixed_Config.Coefficients.Ld.quantized  OutDataTypeStr=FOC_Fixed_Config.Types.Work
  Product : Product  OutDataTypeStr=FOC_Fixed_Config.Types.Work  RndMeth=Convergent  SaturateOnIntegerOverflow=on
  Product1 : Product  OutDataTypeStr=FOC_Fixed_Config.Types.Work  RndMeth=Convergent  SaturateOnIntegerOverflow=on
  Reset_Integral : Switch  Criteria=u2 > Threshold  Threshold=0.5  OutDataTypeStr=FOC_Fixed_Config.Types.Work  RndMeth=Convergent  InputSameDT=off
  Reset_Output : Switch  Criteria=u2 > Threshold  Threshold=0.5  OutDataTypeStr=FOC_Fixed_Config.Types.Work  RndMeth=Convergent  InputSameDT=off
  Reset_Zero : Constant  Value=0  OutDataTypeStr=FOC_Fixed_Config.Types.Work
  Sum : Sum  Inputs=|+-  OutDataTypeStr=FOC_Fixed_Config.Types.Work  AccumDataTypeStr=FOC_Fixed_Config.Types.Work  RndMeth=Convergent  SaturateOnIntegerOverflow=on
  Sum1 : Sum  Inputs=|++  OutDataTypeStr=FOC_Fixed_Config.Types.Work  AccumDataTypeStr=FOC_Fixed_Config.Types.Work  RndMeth=Convergent  SaturateOnIntegerOverflow=on
  x_q_z : UnitDelay  SampleTime=-1
  uq_raw : Outport
  wires:
  Product1/1 -> Sum1/2  "Ed"
  Add1/1 -> Sum1/1
  Gain/1 -> Add2/3  "u_q,aw"
  " "/1 -> Add2/2  "KiTs_q * e_q"
  x_q_z/1 -> Add1/2, Add2/1
  Sum1/1 -> Reset_Output/3
  Add2/1 -> Reset_Integral/3  "x_q_next"
  Reset_Zero/1 -> Reset_Integral/1, Reset_Output/1
  PI_Reset_EN/1 -> Reset_Integral/2, Reset_Output/2
  Reset_Integral/1 -> [x_q_next]
  Reset_Output/1 -> uq_raw/1
  we/1 -> Product1/2
  iq/1 -> Sum/2
  id/1 -> Product/1
  Ld/1 -> Product/2
  Product/1 -> Add/1
  Constant/1 -> Add/2
  Add/1 -> Product1/1
  Sum/1 -> "  "/1, " "/1  "e_q"
  "  "/1 -> Add1/1  "uq_p"
  du_q_z/1 -> [du_q_z]
  [du_q_z] -> Gain/1
  [x_q_next] -> x_q_z/1
  Iq_ref/1 -> Sum/1

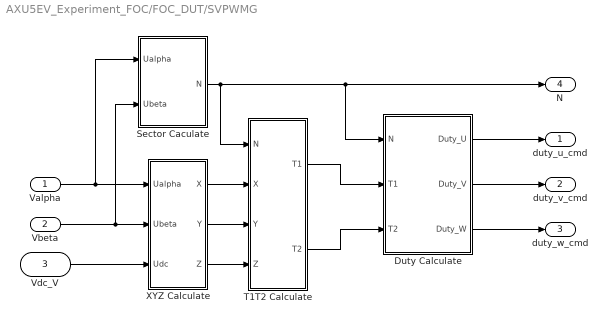
== system AXU5EV_Experiment_FOC/FOC_DUT/SVPWMG ==
  Valpha : Inport
  Vbeta : Inport  Port=2
  Vdc_V : Inport  Port=3
  Duty Calculate : Subsystem  TreatAsAtomicUnit=on  RTWFcnName=Duty_Caculate_Fun
      settings: RTWFcnNameOpts=User specified
  Sector Caculate : Subsystem  TreatAsAtomicUnit=on  RTWFcnName=Sector_Caculate_Fun
      settings: RTWFcnNameOpts=User specified
  T1T2 Calculate : Subsystem  TreatAsAtomicUnit=on  RTWFcnName=T1T2Caculate_Fun
      settings: RTWFcnNameOpts=User specified
  XYZ Calculate : Subsystem  TreatAsAtomicUnit=on  RTWFcnName=XYZ_Caculate_Fun
      settings: RTWFcnNameOpts=User specified
  duty_u_cmd : Outport
  duty_v_cmd : Outport  Port=2
  duty_w_cmd : Outport  Port=3
  "N " : Outport  Port=4
  wires:
  Vbeta/1 -> Sector Caculate/2(Ubeta), XYZ Calculate/2(Ubeta)
  T1T2 Calculate/1(T1) -> Duty Calculate/2(T1)
  Valpha/1 -> Sector Caculate/1(Ualpha), XYZ Calculate/1(Ualpha)
  T1T2 Calculate/2(T2) -> Duty Calculate/3(T2)
  Sector Caculate/1("N ") -> "N "/1, Duty Calculate/1(N), T1T2 Calculate/1(N)
  XYZ Calculate/1(X) -> T1T2 Calculate/2(X)
  XYZ Calculate/2(Y) -> T1T2 Calculate/3(Y)
  XYZ Calculate/3(Z) -> T1T2 Calculate/4(Z)
  Duty Calculate/1(Duty_U) -> duty_u_cmd/1
  Duty Calculate/2(Duty_V) -> duty_v_cmd/1
  Duty Calculate/3(Duty_W) -> duty_w_cmd/1
  Vdc_V/1 -> XYZ Calculate/3(Udc)

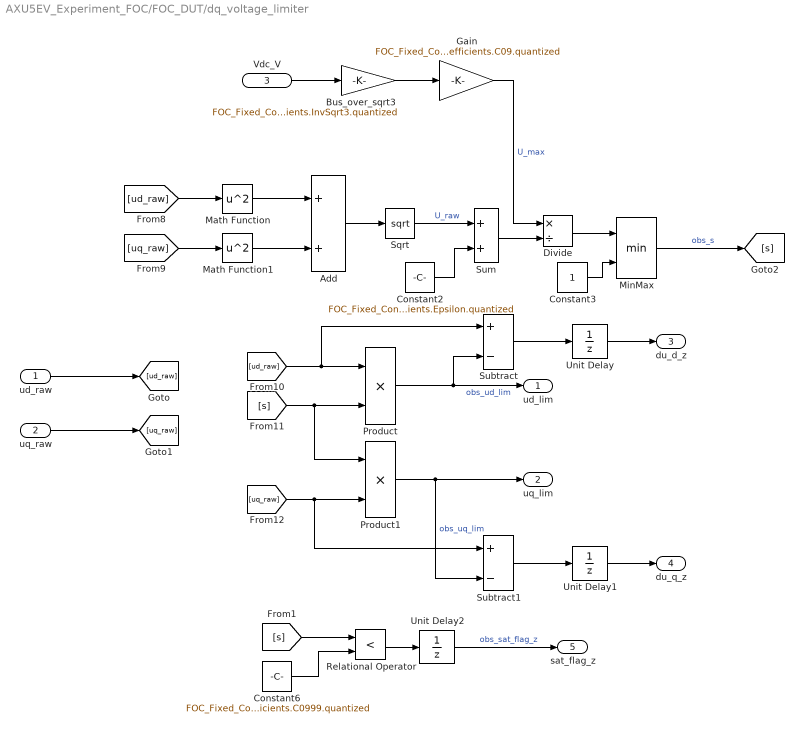
== system AXU5EV_Experiment_FOC/FOC_DUT/dq_voltage_limiter ==
  ud_raw : Inport
  uq_raw : Inport  Port=2
  Vdc_V : Inport  Port=3
  Add : Sum  OutDataTypeStr=FOC_Fixed_Config.Types.Square  AccumDataTypeStr=FOC_Fixed_Config.Types.Square  RndMeth=Convergent  SaturateOnIntegerOverflow=on
  Bus_over_sqrt3 : Gain  Gain=FOC_Fixed_Config.Coefficients.InvSqrt3.quantized  ParamDataTypeStr=FOC_Fixed_Config.Types.Coefficient  OutDataTypeStr=FOC_Fixed_Config.Types.Work  RndMeth=Convergent  SaturateOnIntegerOverflow=on
  Constant2 : Constant  Value=FOC_Fixed_Config.Coefficients.Epsilon.quantized  OutDataTypeStr=FOC_Fixed_Config.Types.Work
  Constant3 : Constant  OutDataTypeStr=FOC_Fixed_Config.Types.Work
  Constant6 : Constant  Value=FOC_Fixed_Config.Coefficients.C0999.quantized  OutDataTypeStr=FOC_Fixed_Config.Types.Work
  Divide : Product  Inputs=*/  OutDataTypeStr=FOC_Fixed_Config.Types.DivideWide  RndMeth=Convergent  SaturateOnIntegerOverflow=on
  Gain : Gain  Gain=FOC_Fixed_Config.Coefficients.C09.quantized  ParamDataTypeStr=FOC_Fixed_Config.Types.Coefficient  OutDataTypeStr=FOC_Fixed_Config.Types.Work  RndMeth=Convergent  SaturateOnIntegerOverflow=on
  Math Function : Math  Operator=square  OutDataTypeStr=FOC_Fixed_Config.Types.Square  RndMeth=Convergent
  Math Function1 : Math  Operator=square  OutDataTypeStr=FOC_Fixed_Config.Types.Square  RndMeth=Convergent
  MinMax : MinMax  Inputs=2  OutDataTypeStr=FOC_Fixed_Config.Types.Work  RndMeth=Convergent  SaturateOnIntegerOverflow=on
  Product : Product  OutDataTypeStr=FOC_Fixed_Config.Types.Work  RndMeth=Convergent  SaturateOnIntegerOverflow=on
  Product1 : Product  OutDataTypeStr=FOC_Fixed_Config.Types.Work  RndMeth=Convergent  SaturateOnIntegerOverflow=on
  Relational Operator : RelationalOperator  Operator=<  OutDataTypeStr=boolean  RndMeth=Convergent  InputSameDT=off
  Sqrt : Sqrt  OutDataTypeStr=FOC_Fixed_Config.Types.Work
  Subtract : Sum  Inputs=+-  OutDataTypeStr=FOC_Fixed_Config.Types.Work  AccumDataTypeStr=FOC_Fixed_Config.Types.Work  RndMeth=Convergent  SaturateOnIntegerOverflow=on
  Subtract1 : Sum  Inputs=+-  OutDataTypeStr=FOC_Fixed_Config.Types.Work  AccumDataTypeStr=FOC_Fixed_Config.Types.Work  RndMeth=Convergent  SaturateOnIntegerOverflow=on
  Sum : Sum  OutDataTypeStr=FOC_Fixed_Config.Types.Work  AccumDataTypeStr=FOC_Fixed_Config.Types.Work  RndMeth=Convergent  SaturateOnIntegerOverflow=on
  Unit Delay : UnitDelay  SampleTime=-1
  Unit Delay1 : UnitDelay  SampleTime=-1
  Unit Delay2 : UnitDelay  SampleTime=-1
  ud_lim : Outport
  uq_lim : Outport  Port=2
  du_d_z : Outport  Port=3
  du_q_z : Outport  Port=4
  sat_flag_z : Outport  Port=5
  wires:
  Sum/1 -> Divide/2
  Constant2/1 -> Sum/2
  Constant3/1 -> MinMax/2
  Add/1 -> Sqrt/1
  Divide/1 -> MinMax/1
  Sqrt/1 -> Sum/1  "U_raw"
  Math Function1/1 -> Add/2
  Math Function/1 -> Add/1
  [uq_raw] -> Math Function1/1
  [ud_raw] -> Math Function/1
  MinMax/1 -> [s]  "obs_s"
  Product1/1 -> uq_lim/1, Subtract1/2  "obs_uq_lim"
  [s] -> Product1/1, Product/2
  [ud_raw] -> Subtract/1, Product/1
  Product/1 -> Subtract/2, ud_lim/1  "obs_ud_lim"
  [uq_raw] -> Subtract1/1, Product1/2
  Subtract/1 -> Unit Delay/1
  Subtract1/1 -> Unit Delay1/1
  ud_raw/1 -> [ud_raw]
  uq_raw/1 -> [uq_raw]
  Unit Delay/1 -> du_d_z/1
  Unit Delay1/1 -> du_q_z/1
  Constant6/1 -> Relational Operator/2
  [s] -> Relational Operator/1
  Relational Operator/1 -> Unit Delay2/1
  Unit Delay2/1 -> sat_flag_z/1  "obs_sat_flag_z"
  Vdc_V/1 -> Bus_over_sqrt3/1
  Bus_over_sqrt3/1 -> Gain/1
  Gain/1 -> Divide/1  "U_max"

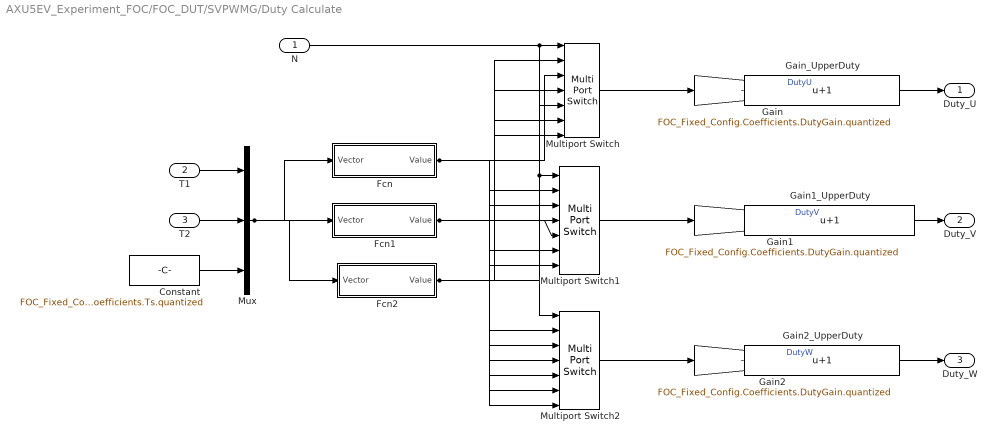
== system AXU5EV_Experiment_FOC/FOC_DUT/SVPWMG/Duty Calculate ==
  N : Inport
  T1 : Inport  Port=2
  T2 : Inport  Port=3
  Constant : Constant  Value=FOC_Fixed_Config.Coefficients.Ts.quantized  OutDataTypeStr=FOC_Fixed_Config.Types.Work
  Fcn : Subsystem
  Fcn1 : Subsystem
  Fcn2 : Subsystem
  Gain : Gain  Gain=FOC_Fixed_Config.Coefficients.DutyGain.quantized  ParamDataTypeStr=FOC_Fixed_Config.Types.Coefficient  OutDataTypeStr=FOC_Fixed_Config.Types.Work  RndMeth=Convergent  SaturateOnIntegerOverflow=on
  Gain1 : Gain  Gain=FOC_Fixed_Config.Coefficients.DutyGain.quantized  ParamDataTypeStr=FOC_Fixed_Config.Types.Coefficient  OutDataTypeStr=FOC_Fixed_Config.Types.Work  RndMeth=Convergent  SaturateOnIntegerOverflow=on
  Gain1_UpperDuty : Bias  Bias=1
  Gain2 : Gain  Gain=FOC_Fixed_Config.Coefficients.DutyGain.quantized  ParamDataTypeStr=FOC_Fixed_Config.Types.Coefficient  OutDataTypeStr=FOC_Fixed_Config.Types.Work  RndMeth=Convergent  SaturateOnIntegerOverflow=on
  Gain2_UpperDuty : Bias  Bias=1
  Gain_UpperDuty : Bias  Bias=1
  Multiport Switch : MultiPortSwitch  Inputs=6  OutDataTypeStr=FOC_Fixed_Config.Types.Work  RndMeth=Convergent  InputSameDT=off
  Multiport Switch1 : MultiPortSwitch  Inputs=6  OutDataTypeStr=FOC_Fixed_Config.Types.Work  RndMeth=Convergent  InputSameDT=off
  Multiport Switch2 : MultiPortSwitch  Inputs=6  OutDataTypeStr=FOC_Fixed_Config.Types.Work  RndMeth=Convergent  InputSameDT=off
  Mux : Mux  Inputs=3
  Duty_U : Outport
  Duty_V : Outport  Port=2
  Duty_W : Outport  Port=3
  wires:
  Gain2_UpperDuty/1 -> Duty_W/1
  Gain2/1 -> Gain2_UpperDuty/1  "DutyW"
  Gain1_UpperDuty/1 -> Duty_V/1
  Gain1/1 -> Gain1_UpperDuty/1  "DutyV"
  Gain_UpperDuty/1 -> Duty_U/1
  Gain/1 -> Gain_UpperDuty/1  "DutyU"
  Mux/1 -> Fcn/1(Vector), Fcn1/1(Vector), Fcn2/1(Vector)
  Constant/1 -> Mux/3
  T2/1 -> Mux/2
  T1/1 -> Mux/1
  Multiport Switch2/1 -> Gain2/1
  Multiport Switch1/1 -> Gain1/1
  Multiport Switch/1 -> Gain/1
  N/1 -> Multiport Switch2/1, Multiport Switch1/1, Multiport Switch/1
  Fcn/1(Value) -> Multiport Switch/3, Multiport Switch/4, Multiport Switch1/6, Multiport Switch2/5, Multiport Switch2/7, Multiport Switch1/2
  Fcn1/1(Value) -> Multiport Switch1/5, Multiport Switch2/3, Multiport Switch2/6, Multiport Switch1/4, Multiport Switch/7, Multiport Switch/2
  Fcn2/1(Value) -> Multiport Switch/5, Multiport Switch/6, Multiport Switch1/3, Multiport Switch1/7, Multiport Switch2/2, Multiport Switch2/4

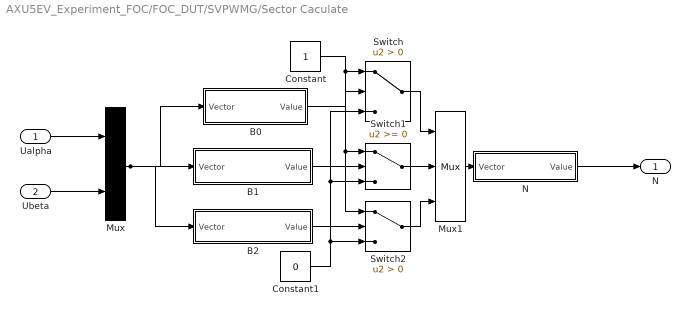
== system AXU5EV_Experiment_FOC/FOC_DUT/SVPWMG/Sector Caculate ==
  Ualpha : Inport
  Ubeta : Inport  Port=2
  B0 : Subsystem
  B1 : Subsystem
  B2 : Subsystem
  Constant : Constant  OutDataTypeStr=uint8
  Constant1 : Constant  Value=0  OutDataTypeStr=uint8
  Mux : Mux  Inputs=2
  Mux1 : Mux  Inputs=3
  N : Subsystem
  Switch : Switch  Criteria=u2 > Threshold  OutDataTypeStr=uint8  RndMeth=Convergent  InputSameDT=off
  Switch1 : Switch  OutDataTypeStr=uint8  RndMeth=Convergent  InputSameDT=off
  Switch2 : Switch  Criteria=u2 > Threshold  OutDataTypeStr=uint8  RndMeth=Convergent  InputSameDT=off
  "N " : Outport  VectorParamsAs1DForOutWhenUnconnected=off
  wires:
  Switch2/1 -> Mux1/3
  Switch/1 -> Mux1/1
  Ualpha/1 -> Mux/1
  Ubeta/1 -> Mux/2
  Mux/1 -> B0/1(Vector), B1/1(Vector), B2/1(Vector)
  Constant/1 -> Switch/1, Switch2/1, Switch1/1
  Constant1/1 -> Switch/3, Switch1/3, Switch2/3
  Switch1/1 -> Mux1/2
  B0/1(Value) -> Switch/2
  B1/1(Value) -> Switch1/2
  B2/1(Value) -> Switch2/2
  Mux1/1 -> N/1(Vector)
  N/1(Value) -> "N "/1

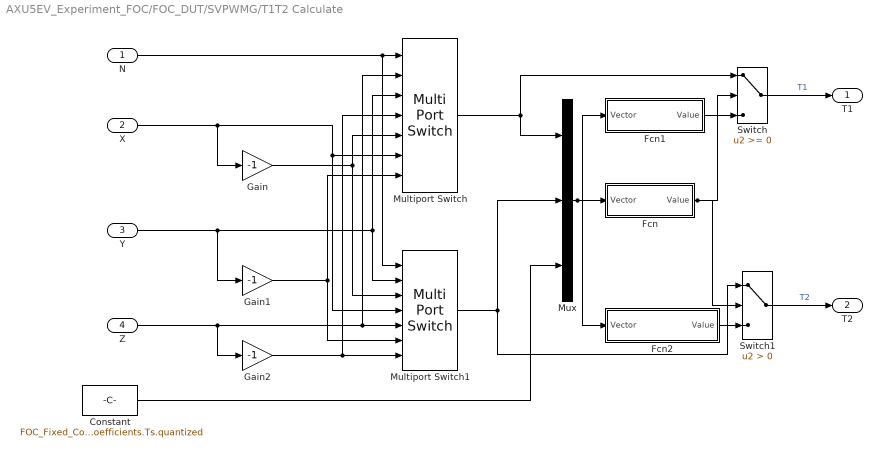
== system AXU5EV_Experiment_FOC/FOC_DUT/SVPWMG/T1T2 Calculate ==
  N : Inport
  X : Inport  Port=2
  Y : Inport  Port=3
  Z : Inport  Port=4
  Constant : Constant  Value=FOC_Fixed_Config.Coefficients.Ts.quantized  OutDataTypeStr=FOC_Fixed_Config.Types.Work
  Fcn : Subsystem
  Fcn1 : Subsystem
  Fcn2 : Subsystem
  Gain : Gain  Gain=-1  ParamDataTypeStr=FOC_Fixed_Config.Types.Coefficient  OutDataTypeStr=FOC_Fixed_Config.Types.Work  RndMeth=Convergent  SaturateOnIntegerOverflow=on
  Gain1 : Gain  Gain=-1  ParamDataTypeStr=FOC_Fixed_Config.Types.Coefficient  OutDataTypeStr=FOC_Fixed_Config.Types.Work  RndMeth=Convergent  SaturateOnIntegerOverflow=on
  Gain2 : Gain  Gain=-1  ParamDataTypeStr=FOC_Fixed_Config.Types.Coefficient  OutDataTypeStr=FOC_Fixed_Config.Types.Work  RndMeth=Convergent  SaturateOnIntegerOverflow=on
  Multiport Switch : MultiPortSwitch  Inputs=6  OutDataTypeStr=FOC_Fixed_Config.Types.Work  RndMeth=Convergent  InputSameDT=off
  Multiport Switch1 : MultiPortSwitch  Inputs=6  OutDataTypeStr=FOC_Fixed_Config.Types.Work  RndMeth=Convergent  InputSameDT=off
  Mux : Mux  Inputs=3
  Switch : Switch  OutDataTypeStr=FOC_Fixed_Config.Types.Work  RndMeth=Convergent  InputSameDT=off
  Switch1 : Switch  Criteria=u2 > Threshold  OutDataTypeStr=FOC_Fixed_Config.Types.Work  RndMeth=Convergent  InputSameDT=off
  T1 : Outport  VectorParamsAs1DForOutWhenUnconnected=off
  T2 : Outport  Port=2  VectorParamsAs1DForOutWhenUnconnected=off
  wires:
  Constant/1 -> Mux/3
  Switch1/1 -> T2/1  "T2"
  Switch/1 -> T1/1  "T1"
  Mux/1 -> Fcn1/1(Vector), Fcn2/1(Vector), Fcn/1(Vector)
  Multiport Switch/1 -> Switch/1, Mux/1
  Multiport Switch1/1 -> Switch1/1, Mux/2
  N/1 -> Multiport Switch/1, Multiport Switch1/1
  Y/1 -> Multiport Switch/3, Multiport Switch1/2, Gain1/1
  Z/1 -> Multiport Switch1/5, Multiport Switch/2, Gain2/1
  X/1 -> Gain/1, Multiport Switch/6, Multiport Switch1/4
  Gain/1 -> Multiport Switch1/3, Multiport Switch/5
  Gain2/1 -> Multiport Switch/4, Multiport Switch1/7
  Gain1/1 -> Multiport Switch1/6, Multiport Switch/7
  Fcn1/1(Value) -> Switch/3
  Fcn2/1(Value) -> Switch1/3
  Fcn/1(Value) -> Switch/2, Switch1/2

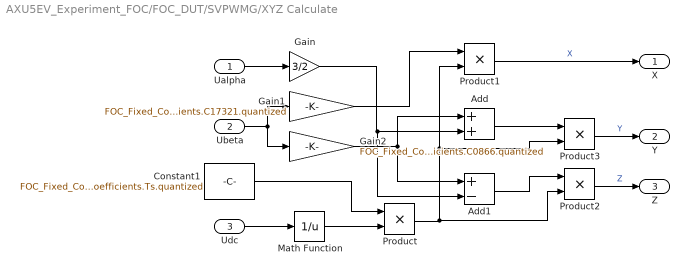
== system AXU5EV_Experiment_FOC/FOC_DUT/SVPWMG/XYZ Calculate ==
  Ualpha : Inport
  Ubeta : Inport  Port=2
  Udc : Inport  Port=3
  Add : Sum  OutDataTypeStr=FOC_Fixed_Config.Types.Work  AccumDataTypeStr=FOC_Fixed_Config.Types.Work  RndMeth=Convergent  SaturateOnIntegerOverflow=on
  Add1 : Sum  Inputs=+-  OutDataTypeStr=FOC_Fixed_Config.Types.Work  AccumDataTypeStr=FOC_Fixed_Config.Types.Work  RndMeth=Convergent  SaturateOnIntegerOverflow=on
  Constant1 : Constant  Value=FOC_Fixed_Config.Coefficients.Ts.quantized  OutDataTypeStr=FOC_Fixed_Config.Types.Work
  Gain : Gain  Gain=3/2  ParamDataTypeStr=FOC_Fixed_Config.Types.Coefficient  OutDataTypeStr=FOC_Fixed_Config.Types.Work  RndMeth=Convergent  SaturateOnIntegerOverflow=on
  Gain1 : Gain  Gain=FOC_Fixed_Config.Coefficients.C17321.quantized  ParamDataTypeStr=FOC_Fixed_Config.Types.Coefficient  OutDataTypeStr=FOC_Fixed_Config.Types.Work  RndMeth=Convergent  SaturateOnIntegerOverflow=on
  Gain2 : Gain  Gain=FOC_Fixed_Config.Coefficients.C0866.quantized  ParamDataTypeStr=FOC_Fixed_Config.Types.Coefficient  OutDataTypeStr=FOC_Fixed_Config.Types.Work  RndMeth=Convergent  SaturateOnIntegerOverflow=on
  Math Function : Math  Operator=reciprocal  OutDataTypeStr=FOC_Fixed_Config.Types.Work  RndMeth=Convergent
  Product{,1..3} (4 alike) : Product  OutDataTypeStr=FOC_Fixed_Config.Types.Work  RndMeth=Convergent  SaturateOnIntegerOverflow=on
  X : Outport
  Y : Outport  Port=2
  Z : Outport  Port=3
  wires:
  Ualpha/1 -> Gain/1
  Udc/1 -> Math Function/1
  Math Function/1 -> Product/2
  Ubeta/1 -> Gain2/1, Gain1/1
  Gain1/1 -> Product1/1
  Product/1 -> Product2/2, Product3/2, Product1/2
  Gain2/1 -> Add/1, Add1/1
  Gain/1 -> Add1/2, Add/2
  Product1/1 -> X/1  "X"
  Add/1 -> Product3/1
  Add1/1 -> Product2/1
  Product2/1 -> Z/1  "Z"
  Product3/1 -> Y/1  "Y"
  Constant1/1 -> Product/1

== system AXU5EV_Experiment_FOC/FOC_DUT/SVPWMG/Duty Calculate/Fcn ==
  Vector : Inport
  Combination : Sum  Inputs=+--  OutDataTypeStr=FOC_Fixed_Config.Types.Work  AccumDataTypeStr=FOC_Fixed_Config.Types.Work  RndMeth=Convergent  SaturateOnIntegerOverflow=on
  Elements : Demux  Outputs=3
  Quarter : Gain  Gain=.25  ParamDataTypeStr=FOC_Fixed_Config.Types.Coefficient  OutDataTypeStr=FOC_Fixed_Config.Types.Work  RndMeth=Convergent  SaturateOnIntegerOverflow=on
  Value : Outport
  wires:
  Vector/1 -> Elements/1
  Elements/2 -> Combination/3
  Elements/1 -> Combination/2
  Elements/3 -> Combination/1
  Combination/1 -> Quarter/1
  Quarter/1 -> Value/1

== system AXU5EV_Experiment_FOC/FOC_DUT/SVPWMG/Duty Calculate/Fcn1 ==
  Vector : Inport
  Combination : Sum  Inputs=++-  OutDataTypeStr=FOC_Fixed_Config.Types.Work  AccumDataTypeStr=FOC_Fixed_Config.Types.Work  RndMeth=Convergent  SaturateOnIntegerOverflow=on
  Elements : Demux  Outputs=3
  Quarter : Gain  Gain=.25  ParamDataTypeStr=FOC_Fixed_Config.Types.Coefficient  OutDataTypeStr=FOC_Fixed_Config.Types.Work  RndMeth=Convergent  SaturateOnIntegerOverflow=on
  Value : Outport
  wires:
  Vector/1 -> Elements/1
  Elements/1 -> Combination/2
  Elements/3 -> Combination/1
  Elements/2 -> Combination/3
  Combination/1 -> Quarter/1
  Quarter/1 -> Value/1

== system AXU5EV_Experiment_FOC/FOC_DUT/SVPWMG/Duty Calculate/Fcn2 ==
  Vector : Inport
  Combination : Sum  Inputs=+++  OutDataTypeStr=FOC_Fixed_Config.Types.Work  AccumDataTypeStr=FOC_Fixed_Config.Types.Work  RndMeth=Convergent  SaturateOnIntegerOverflow=on
  Elements : Demux  Outputs=3
  Quarter : Gain  Gain=.25  ParamDataTypeStr=FOC_Fixed_Config.Types.Coefficient  OutDataTypeStr=FOC_Fixed_Config.Types.Work  RndMeth=Convergent  SaturateOnIntegerOverflow=on
  Value : Outport
  wires:
  Vector/1 -> Elements/1
  Elements/1 -> Combination/3
  Elements/3 -> Combination/1
  Elements/2 -> Combination/2
  Combination/1 -> Quarter/1
  Quarter/1 -> Value/1

== system AXU5EV_Experiment_FOC/FOC_DUT/SVPWMG/Sector Caculate/B0 ==
  Vector : Inport
  Elements : Demux  Outputs=2
  Unused_Vector_Element : Terminator
  Value : Outport
  wires:
  Vector/1 -> Elements/1
  Elements/2 -> Value/1
  Elements/1 -> Unused_Vector_Element/1

== system AXU5EV_Experiment_FOC/FOC_DUT/SVPWMG/Sector Caculate/B1 ==
  Vector : Inport
  Alpha0866 : Gain  Gain=FOC_Fixed_Config.Coefficients.C0866.quantized  ParamDataTypeStr=FOC_Fixed_Config.Types.Coefficient  OutDataTypeStr=FOC_Fixed_Config.Types.Work  RndMeth=Convergent  SaturateOnIntegerOverflow=on
  Beta05 : Gain  Gain=0.5  ParamDataTypeStr=FOC_Fixed_Config.Types.Coefficient  OutDataTypeStr=FOC_Fixed_Config.Types.Work  RndMeth=Convergent  SaturateOnIntegerOverflow=on
  Elements : Demux  Outputs=2
  Projection : Sum  Inputs=+-  OutDataTypeStr=FOC_Fixed_Config.Types.Work  AccumDataTypeStr=FOC_Fixed_Config.Types.Work  RndMeth=Convergent  SaturateOnIntegerOverflow=on
  Value : Outport
  wires:
  Vector/1 -> Elements/1
  Elements/1 -> Alpha0866/1
  Elements/2 -> Beta05/1
  Alpha0866/1 -> Projection/1
  Beta05/1 -> Projection/2
  Projection/1 -> Value/1

== system AXU5EV_Experiment_FOC/FOC_DUT/SVPWMG/Sector Caculate/B2 ==
  Vector : Inport
  Alpha0866 : Gain  Gain=FOC_Fixed_Config.Coefficients.C0866.quantized  ParamDataTypeStr=FOC_Fixed_Config.Types.Coefficient  OutDataTypeStr=FOC_Fixed_Config.Types.Work  RndMeth=Convergent  SaturateOnIntegerOverflow=on
  Beta05 : Gain  Gain=0.5  ParamDataTypeStr=FOC_Fixed_Config.Types.Coefficient  OutDataTypeStr=FOC_Fixed_Config.Types.Work  RndMeth=Convergent  SaturateOnIntegerOverflow=on
  Elements : Demux  Outputs=2
  Projection : Sum  Inputs=--  OutDataTypeStr=FOC_Fixed_Config.Types.Work  AccumDataTypeStr=FOC_Fixed_Config.Types.Work  RndMeth=Convergent  SaturateOnIntegerOverflow=on
  Value : Outport
  wires:
  Vector/1 -> Elements/1
  Elements/2 -> Beta05/1
  Elements/1 -> Alpha0866/1
  Alpha0866/1 -> Projection/1
  Beta05/1 -> Projection/2
  Projection/1 -> Value/1

== system AXU5EV_Experiment_FOC/FOC_DUT/SVPWMG/Sector Caculate/N ==
  Vector : Inport  OutDataTypeStr=uint8
  Elements : Demux  Outputs=3
  Four : Gain  Gain=4  ParamDataTypeStr=uint8  OutDataTypeStr=uint8  RndMeth=Convergent  SaturateOnIntegerOverflow=on
  SectorNumber : Sum  Inputs=+++  OutDataTypeStr=uint8  AccumDataTypeStr=uint8  RndMeth=Convergent  SaturateOnIntegerOverflow=on
  Two : Gain  Gain=2  ParamDataTypeStr=uint8  OutDataTypeStr=uint8  RndMeth=Convergent  SaturateOnIntegerOverflow=on
  Value : Outport  OutDataTypeStr=uint8
  wires:
  Vector/1 -> Elements/1
  SectorNumber/1 -> Value/1
  Elements/1 -> SectorNumber/3
  Elements/3 -> Four/1
  Elements/2 -> Two/1
  Four/1 -> SectorNumber/1
  Two/1 -> SectorNumber/2

== system AXU5EV_Experiment_FOC/FOC_DUT/SVPWMG/T1T2 Calculate/Fcn ==
  Vector : Inport
  Combination : Sum  Inputs=+--  OutDataTypeStr=FOC_Fixed_Config.Types.Work  AccumDataTypeStr=FOC_Fixed_Config.Types.Work  RndMeth=Convergent  SaturateOnIntegerOverflow=on
  Elements : Demux  Outputs=3
  Value : Outport
  wires:
  Vector/1 -> Elements/1
  Elements/1 -> Combination/3
  Elements/2 -> Combination/2
  Elements/3 -> Combination/1
  Combination/1 -> Value/1

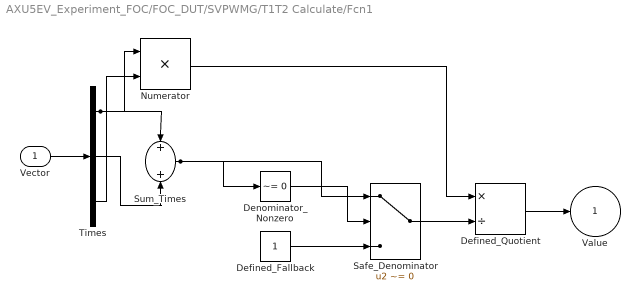
== system AXU5EV_Experiment_FOC/FOC_DUT/SVPWMG/T1T2 Calculate/Fcn1 ==
  Vector : Inport
  Defined_Fallback : Constant  OutDataTypeStr=FOC_Fixed_Config.Types.Work
  Defined_Quotient : Product  Inputs=*/  OutDataTypeStr=FOC_Fixed_Config.Types.Work  RndMeth=Convergent  SaturateOnIntegerOverflow=on
  Denominator_Nonzero : simulink/Logic and Bit Operations/Compare To Zero  relop=~=  OutDataTypeStr=boolean
  Numerator : Product  Inputs=**  OutDataTypeStr=FOC_Fixed_Config.Types.Work  RndMeth=Convergent  SaturateOnIntegerOverflow=on
  Safe_Denominator : Switch  Criteria=u2 ~= 0  OutDataTypeStr=FOC_Fixed_Config.Types.Work  RndMeth=Convergent  InputSameDT=off
  Sum_Times : Sum  OutDataTypeStr=FOC_Fixed_Config.Types.Work  AccumDataTypeStr=FOC_Fixed_Config.Types.Work  RndMeth=Convergent  SaturateOnIntegerOverflow=on
  Times : Demux  Outputs=3
  Value : Outport
  wires:
  Times/1 -> Sum_Times/1, Numerator/1
  Vector/1 -> Times/1
  Numerator/1 -> Defined_Quotient/1
  Times/2 -> Sum_Times/2
  Times/3 -> Numerator/2
  Sum_Times/1 -> Safe_Denominator/1, Denominator_Nonzero/1
  Denominator_Nonzero/1 -> Safe_Denominator/2
  Defined_Fallback/1 -> Safe_Denominator/3
  Safe_Denominator/1 -> Defined_Quotient/2
  Defined_Quotient/1 -> Value/1

== system AXU5EV_Experiment_FOC/FOC_DUT/SVPWMG/T1T2 Calculate/Fcn2 ==
  Vector : Inport
  Defined_Fallback : Constant  OutDataTypeStr=FOC_Fixed_Config.Types.Work
  Defined_Quotient : Product  Inputs=*/  OutDataTypeStr=FOC_Fixed_Config.Types.Work  RndMeth=Convergent  SaturateOnIntegerOverflow=on
  Denominator_Nonzero : simulink/Logic and Bit Operations/Compare To Zero  relop=~=  OutDataTypeStr=boolean
  Numerator : Product  Inputs=**  OutDataTypeStr=FOC_Fixed_Config.Types.Work  RndMeth=Convergent  SaturateOnIntegerOverflow=on
  Safe_Denominator : Switch  Criteria=u2 ~= 0  OutDataTypeStr=FOC_Fixed_Config.Types.Work  RndMeth=Convergent  InputSameDT=off
  Sum_Times : Sum  OutDataTypeStr=FOC_Fixed_Config.Types.Work  AccumDataTypeStr=FOC_Fixed_Config.Types.Work  RndMeth=Convergent  SaturateOnIntegerOverflow=on
  Times : Demux  Outputs=3
  Value : Outport
  wires:
  Times/3 -> Numerator/2
  Vector/1 -> Times/1
  Times/1 -> Sum_Times/1
  Times/2 -> Sum_Times/2, Numerator/1
  Numerator/1 -> Defined_Quotient/1
  Sum_Times/1 -> Safe_Denominator/1, Denominator_Nonzero/1
  Denominator_Nonzero/1 -> Safe_Denominator/2
  Defined_Fallback/1 -> Safe_Denominator/3
  Safe_Denominator/1 -> Defined_Quotient/2
  Defined_Quotient/1 -> Value/1
